simulink model "untitled"  (R2023a)
settings: Solver=VariableStepAuto  StartTime=0.0  StopTime=10.0  RelTol=1e-3
settings Model: Creator=Administrator  LastModifiedBy=Administrator
settings SolverCC: AlgebraicLoopSolver=TrustRegion
settings DataIOCC: LimitDataPoints=on  SaveOutput=off  SaveTime=off
settings OptimizationCC: BlockReduction=off  BooleanDataType=off  LifeSpan=inf
settings DebuggingCC: SaveWithParameterizedLinksMsg=none  UnderspecifiedInitializationDetection=Classic  MergeDetectMultiDrivingBlocksExec=none  SignalResolutionControl=TryResolveAllWithWarning  UnconnectedInputMsg=warning  UnconnectedOutputMsg=warning  UnconnectedLineMsg=warning  AllowSymbolicDim=off  SFUnexpectedBacktrackingDiag=warning  SFNoUnconditionalDefaultTransitionDiag=warning  SFExecutionAtInitializationDiag=none  ArithmeticOperatorsInVariantConditions=warning
settings HardwareCC: TargetUnknown=on
settings ModelReferenceCC: EnableRefExpFcnMdlSchedulingChecks=on
settings SFSimCC: SimUseLocalCustomCode=off  CustomCodeUndefinedFunction=UseInterfaceOnly
settings RTWCC: RTWUseLocalCustomCode=off
settings CodeAppCC: StateflowObjectComments=on
settings GRTTargetCC: TargetLangStandard=C89/C90 (ANSI)

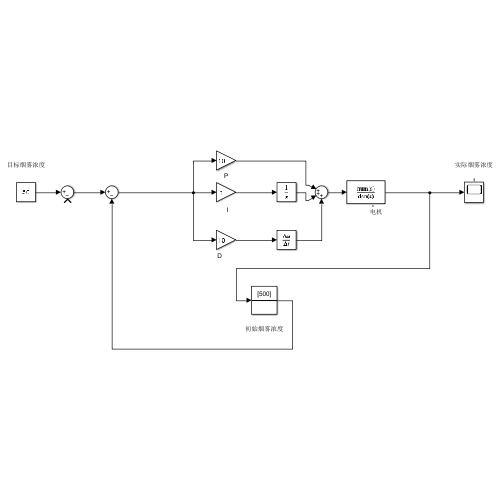
[thumbnail: Simulink's stored preview of the top-level diagram]
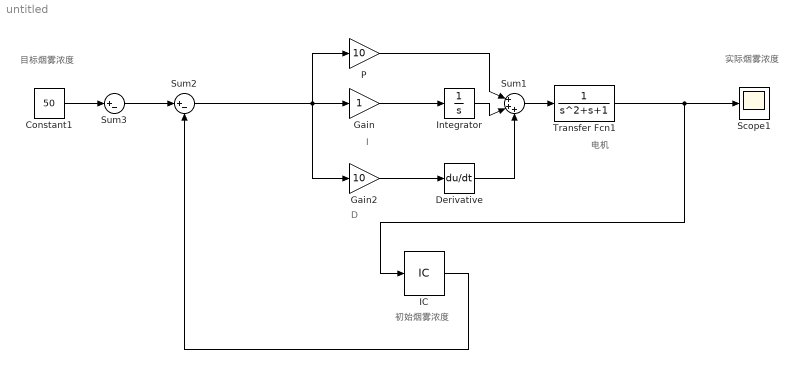
== system untitled ==
  note: 实际烟雾浓度
  note: 电机
  note: D
  note: I
  note: 目标烟雾浓度
  note: 初始烟雾浓度
  Constant1 : Constant  Value=50
  Derivative : Derivative
  Gain : Gain
  Gain2 : Gain  Gain=10
  IC : InitialCondition  Value=500
  Integrator : Integrator
  P : Gain  Gain=10
  Scope1 : Scope
  Sum1 : Sum  Inputs=|+++
  Sum2 : Sum  Inputs=|+-
  Sum3 : Sum  Inputs=|+-
  Transfer Fcn1 : TransferFcn  Denominator=[1 1 1]  AbsoluteTolerance=100
  wires:
  Gain/1 -> Integrator/1
  Gain2/1 -> Derivative/1
  Sum1/1 -> Transfer Fcn1/1
  Derivative/1 -> Sum1/3
  Integrator/1 -> Sum1/2
  P/1 -> Sum1/1
  Transfer Fcn1/1 -> IC/1, Scope1/1
  Sum2/1 -> Gain2/1, P/1, Gain/1
  Constant1/1 -> Sum3/1
  Sum3/1 -> Sum2/1
  IC/1 -> Sum2/2
